simulink model "Main_SpeedOptimisedVersionTannenweg"  (R2024b)
settings: Solver=ode15s  StartTime=0.0  StopTime=3600*2  FixedStep=0.1  RelTol=0.001
model workspace (MAT data in the model file):
  Ti = 5
  fa = 0.00071
  fd = 0.03
  ips = 36
  ma = 0.0013
  md = 0.04
  roomarea1 = 20
  s = 15
libraries: fl_lib x1434, nesl_utility x105, SimscapeFluids_lib x35
(part 1 of 22)
settings Model: SimulationMode=accelerator  Creator=ferdi  LastModifiedBy=ferdi
settings SolverCC: MaxConsecutiveMinStep=5  ZeroCrossControl=EnableAll

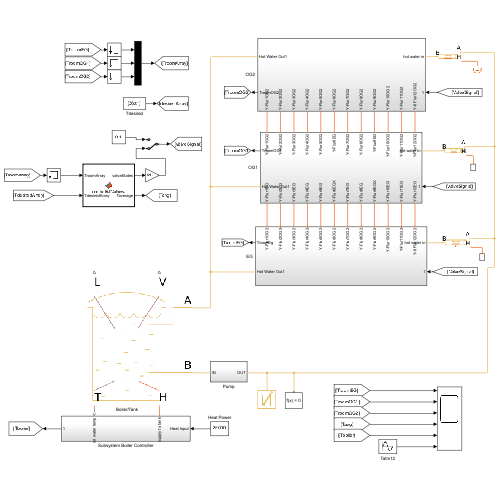
[thumbnail: Simulink's stored preview of the top-level diagram]
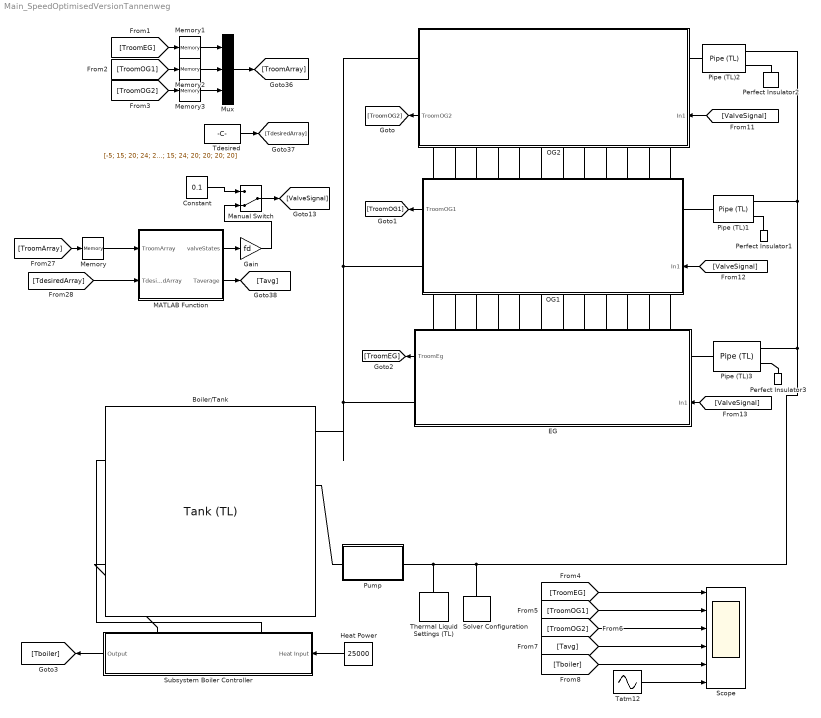
== system Main_SpeedOptimisedVersionTannenweg ==
  Boiler/Tank : SimscapeFluids_lib/Thermal Liquid/Tanks & Accumulators/Tank (TL)  num_inlet=fluids.thermal_liquid.tanks_accumulators.enum.NumInlet.Two  pressure_spec=fluids.thermal_liquid.tanks_accumulators.enum.TankPressureSpec.Atmospheric  tank_pressure=0.101325 MPa  volume_spec=fluids.thermal_liquid.tanks_accumulators.enum.TankVolumeSpec.Constant  tank_area=5 m^2  level_TLU=[0, 3, 5] m  volume_TLU=[0, 4, 6] m^3  inlet_height_A=0.1 m  inlet_area_A=0.01 m^2  inlet_heights_AB=[.1, .1] m  inlet_areas_AB=[ma, ma] m^2  inlet_heights_ABC=[.1, .1, .1] m  inlet_areas_ABC=[.01, .01, .01] m^2  inlet_heights_ABCD=0.1 * ones(1, 4) m  inlet_areas_ABCD=0.01 * ones(1, 4) m^2  inlet_heights_ABCDE=0.1 * ones(1, 5) m  inlet_areas_ABCDE=0.01 * ones(1, 5) m^2  inlet_heights_ABCDEF=0.1 * ones(1, 6) m  inlet_areas_ABCDEF=0.01 * ones(1, 6) m^2  level_check=simscape.enum.assert.action.error  capacity_check=simscape.enum.assert.action.none  max_capacity=10 m^3  g=9.81 m/s^2  level_specify=off  level_priority=High  level=5 m  level_nominal_specify=on  level_nominal_value=5  level_nominal_unit=m  volume_specify=on  volume_priority=None  volume=25 m^3  volume_nominal_specify=on  volume_nominal_value=27  volume_nominal_unit=m^3  mass_specify=on  mass_priority=None  mass=25000 kg  mass_nominal_specify=off  mass_nominal_value=1  mass_nominal_unit=kg  T_I_specify=on  T_I_priority=High  T_I=55 degC  T_I_nominal_specify=off  T_I_nominal_value=1  T_I_nominal_unit=K
      settings: InternalSimscapePortConfiguration="{\"Bottom\":[{\"id\":\"H\",\"label\":\"H\",\"type\":\"foundation.thermal.thermal\"},{\"id\":\"T_out\",\"label\":\"T\",\"type\":\"output\"}],\"Left\":[{\"id\":\"A\",\"label\":\"A\",\"type\":\"foundation.thermal_liquid.thermal_liquid\"},{\"id\":\"B\",\"label\":\"B\",\"type\":\"foundation.thermal_liquid.thermal_liquid\"}],\"Right\":[],\"Top\":[{\"id\":\"V_out\",\"label\":\"V\",\"type\":\"output\"},{\"id\":\"L_out\",\"label\":\"L\",\"type\":\"output\"}]}"
  Constant : Constant  Value=0.1
  EG : Subsystem
      settings: PortSchema="{\"entries\":[{\"content\":{\"sides\":[{\"content\":{\"connectorIds\":[\"In1\",\"LConn1\"]},\"type\":\"ConnectorPlacement.EquallySpacedRectSide\",\"uuid\":\"2656af94-fbaa-4cdb-8b28-cfd3398b16ef\"},{\"content\":{\"connectorIds\":[\"RConn1\",\"Out1\"],\"side\":\"RIGHT\"},\"type\":\"ConnectorPlacement.EquallySpacedRectSide\",\"uuid\":\"da923e50-de3a-407d-b440-bba41caa8d09\"},{\"content\":{\"side\":\"TOP\"},\"type\":\"ConnectorPlacement.EquallySpacedRectSide\",\"uuid\":\"d00b7d3b-fad0-43e7-8322-d8df48fa7e08\"},{\"content\":{\"connectorIds\":[\"RConn2\",\"RConn3\",\"RConn4\",\"RConn5\",\"RConn6\",\"RConn7\",\"RConn8\",\"RConn9\",\"RConn10\",\"RConn11\",\"RConn12\",\"RConn13\"],\"side\":\"BOTTOM\"},\"type\":\"ConnectorPlacement.EquallySpacedRectSide\",\"uuid\":\"2d6cf44f-790a-4efb-a1e3-b38be23d7dad\"}]},\"type\":\"ConnectorPlacement.EquallySpacedConnector\",\"uuid\":\"43b409cf-1277-4d86-ba4e-16516e35aeb3\"}],\"packageUris\":[\"http://schema.mathworks.com/mf0/Connector/R2020b\"],\"version\":\"1.0\"}"
  Gain : Gain  Gain=fd
  Heat Power : Constant  Value=25000
  MATLAB Function : MATLAB Function  TreatAsAtomicUnit=on
  Manual Switch : ManualSwitch  CurrentSetting=0
  Memory{,1..3} (4 alike) : Memory
  Mux : Mux  Inputs=3
  OG1 : Subsystem
      settings: PortSchema="{\"entries\":[{\"content\":{\"sides\":[{\"content\":{\"connectorIds\":[\"In1\",\"LConn1\"]},\"type\":\"ConnectorPlacement.EquallySpacedRectSide\",\"uuid\":\"2656af94-fbaa-4cdb-8b28-cfd3398b16ef\"},{\"content\":{\"connectorIds\":[\"RConn1\",\"Out1\"],\"side\":\"RIGHT\"},\"type\":\"ConnectorPlacement.EquallySpacedRectSide\",\"uuid\":\"da923e50-de3a-407d-b440-bba41caa8d09\"},{\"content\":{\"connectorIds\":[\"LConn2\",\"LConn3\",\"LConn4\",\"LConn5\",\"LConn6\",\"LConn7\",\"LConn8\",\"LConn9\",\"LConn10\",\"LConn11\",\"LConn12\",\"LConn13\"],\"side\":\"TOP\"},\"type\":\"ConnectorPlacement.EquallySpacedRectSide\",\"uuid\":\"d00b7d3b-fad0-43e7-8322-d8df48fa7e08\"},{\"content\":{\"connectorIds\":[\"RConn2\",\"RConn3\",\"RConn4\",\"RConn5\",\"RConn6\",\"RConn7\",\"RConn8\",\"RConn9\",\"RConn10\",\"RConn11\",\"RConn12\",\"RConn13\"],\"side\":\"BOTTOM\"},\"type\":\"ConnectorPlacement.EquallySpacedRectSide\",\"uuid\":\"2d6cf44f-790a-4efb-a1e3-b38be23d7dad\"}]},\"type\":\"ConnectorPlacement.EquallySpacedConnector\",\"uuid\":\"43b409cf-1277-4d86-ba4e-16516e35aeb3\"}],\"packageUris\":[\"http://schema.mathworks.com/mf0/Connector/R2020b\"],\"version\":\"1.0\"}"
  OG2 : Subsystem
      settings: PortSchema="{\"entries\":[{\"content\":{\"sides\":[{\"content\":{\"connectorIds\":[\"LConn1\",\"In1\"]},\"type\":\"ConnectorPlacement.EquallySpacedRectSide\",\"uuid\":\"2656af94-fbaa-4cdb-8b28-cfd3398b16ef\"},{\"content\":{\"connectorIds\":[\"RConn1\",\"Out1\"],\"side\":\"RIGHT\"},\"type\":\"ConnectorPlacement.EquallySpacedRectSide\",\"uuid\":\"da923e50-de3a-407d-b440-bba41caa8d09\"},{\"content\":{\"side\":\"TOP\"},\"type\":\"ConnectorPlacement.EquallySpacedRectSide\",\"uuid\":\"d00b7d3b-fad0-43e7-8322-d8df48fa7e08\"},{\"content\":{\"connectorIds\":[\"RConn2\",\"RConn3\",\"RConn4\",\"RConn5\",\"RConn6\",\"RConn7\",\"RConn8\",\"RConn9\",\"RConn10\",\"RConn11\",\"RConn12\",\"RConn13\"],\"side\":\"BOTTOM\"},\"type\":\"ConnectorPlacement.EquallySpacedRectSide\",\"uuid\":\"2d6cf44f-790a-4efb-a1e3-b38be23d7dad\"}]},\"type\":\"ConnectorPlacement.EquallySpacedConnector\",\"uuid\":\"43b409cf-1277-4d86-ba4e-16516e35aeb3\"}],\"packageUris\":[\"http://schema.mathworks.com/mf0/Connector/R2020b\"],\"version\":\"1.0\"}"
  Perfect Insulator1 : fl_lib/Thermal/Thermal Elements/Perfect Insulator  T_specify=off  T_priority=None  T=293.15 K  T_nominal_specify=off  T_nominal_value=1  T_nominal_unit=K
  Perfect Insulator2 : fl_lib/Thermal/Thermal Elements/Perfect Insulator  T_specify=off  T_priority=None  T=293.15 K  T_nominal_specify=off  T_nominal_value=1  T_nominal_unit=K
  Perfect Insulator3 : fl_lib/Thermal/Thermal Elements/Perfect Insulator  T_specify=off  T_priority=None  T=293.15 K  T_nominal_specify=off  T_nominal_value=1  T_nominal_unit=K
  Pipe (TL)1 : fl_lib/Thermal Liquid/Elements/Pipe (TL)  length=4.8 m  area=ma m^2  Dh=md m  length_add=1 m  roughness=15e-6 m  Re_lam=2000  Re_tur=4000  shape_factor=64  Nu_lam=3.66  dynamic_compressibility=true  inertia=false  p0=0.101325 MPa  T0=293.15 K  mdot0=0 kg/s
  Pipe (TL)2 : fl_lib/Thermal Liquid/Elements/Pipe (TL)  length=7.6 m  area=ma m^2  Dh=md m  length_add=1 m  roughness=15e-6 m  Re_lam=2000  Re_tur=4000  shape_factor=64  Nu_lam=3.66  dynamic_compressibility=true  inertia=false  p0=0.101325 MPa  T0=293.15 K  mdot0=0 kg/s
  Pipe (TL)3 : fl_lib/Thermal Liquid/Elements/Pipe (TL)  length=2 m  area=ma m^2  Dh=md m  length_add=1 m  roughness=15e-6 m  Re_lam=2000  Re_tur=4000  shape_factor=64  Nu_lam=3.66  dynamic_compressibility=true  inertia=false  p0=0.101325 MPa  T0=293.15 K  mdot0=0 kg/s
  Pump : Subsystem
      settings: PortSchema="{\"entries\":[{\"content\":{\"sides\":[{\"content\":{},\"type\":\"ConnectorPlacement.EquallySpacedRectSide\",\"uuid\":\"6c4af18d-f8fe-44c2-baba-c678dedb7514\"},{\"content\":{\"side\":\"RIGHT\"},\"type\":\"ConnectorPlacement.EquallySpacedRectSide\",\"uuid\":\"e67d3007-1da7-46b5-b3e8-302f65e107ea\"},{\"content\":{\"connectorIds\":[\"LConn1\"],\"side\":\"TOP\"},\"type\":\"ConnectorPlacement.EquallySpacedRectSide\",\"uuid\":\"e390c6ba-3993-4bdd-a4fa-a3ffec9d74f1\"},{\"content\":{\"connectorIds\":[\"RConn1\"],\"side\":\"BOTTOM\"},\"type\":\"ConnectorPlacement.EquallySpacedRectSide\",\"uuid\":\"a62ac90e-623e-483b-9a51-1fd62e714745\"}]},\"type\":\"ConnectorPlacement.EquallySpacedConnector\",\"uuid\":\"b6a4287e-aed5-4256-ab6a-ea8ae0115076\"}],\"packageUris\":[\"http://schema.mathworks.com/mf0/Connector/R2020b\"],\"version\":\"1.0\"}"
  Scope : Scope  NumInputPorts=6
  Solver Configuration : nesl_utility/Solver Configuration  PhysicalDomain=network_engine_domain  SubClassName=solver  LeftPortType=input  RightPortType=generic  Tones=[]  Harmonics=[]  SimulateNoise=off  Profile=off  UseLocalSampling=off  EnableSwitchedLinearOptims=on  FrequencyDomain=off  UseCCode=off  RelTol=0.001  AbsTol=0.001  MinStep=1e-09  ToWorkspace=off  RevertToSquareIcSolve=off  NumHomotopyIterations=100  PhasorMode=off  PhasorModeNumHarmonics=1  ConsistencySolver=NEWTON_XTOL_AFTER_FTOL  IndexReductionMethod=DerivativeReplacement  DoDC=off  ResidualTolerance=1e-09  ConsistencyTolSource=GLOBAL  ConsistencyAbsTol=0.001  ConsistencyRelTol=0.001  ConsistencyTolFactor=0.001  UseLocalSolver=off  LocalSolverChoice=NE_BACKWARD_EULER_ADVANCER  ResolveIndetEquations=on  FunctionEvalNumThread=1  LocalSolverSampleTime=0.001  DoFixedCost=off  MaxNonlinIter=3  MaxModeIter=2  ComputeImpulses=off  ImpulseIterations=2  LinearAlgebra=auto  LinearAlgebraNumThread=0  EquationFormulation=NE_TIME_EF  DelaysMemoryBudget=1024  AutomaticFiltering=on  FilteringTimeConstant=0.001  PartitionStorageMethod=AS_NEEDED  PartitionMemoryBudget=1024  PartitionMethod=ROBUST  MultibodyUseLocalSolver=off  MultibodyLocalSolverChoice=ODE1  MultibodyLocalSolverSampleTime=0.001
  Subsystem Boiler Controller : Subsystem
      settings: PortSchema="{\"entries\":[{\"content\":{\"sides\":[{\"content\":{\"connectorIds\":[\"In1\"]},\"type\":\"ConnectorPlacement.EquallySpacedRectSide\",\"uuid\":\"e7750da8-9cb3-4133-899c-c72a77ff6dd9\"},{\"content\":{\"connectorIds\":[\"Out1\"],\"side\":\"RIGHT\"},\"type\":\"ConnectorPlacement.EquallySpacedRectSide\",\"uuid\":\"07247844-436f-42d1-bf44-41b0acb7a571\"},{\"content\":{\"connectorIds\":[\"LConn1\",\"LConn2\"],\"side\":\"TOP\"},\"type\":\"ConnectorPlacement.EquallySpacedRectSide\",\"uuid\":\"d71ce214-d117-4844-8b18-b77bcc45f26b\"},{\"content\":{\"side\":\"BOTTOM\"},\"type\":\"ConnectorPlacement.EquallySpacedRectSide\",\"uuid\":\"a67a4664-f3b4-445e-bf57-56add1a19a7b\"}]},\"type\":\"ConnectorPlacement.EquallySpacedConnector\",\"uuid\":\"1154f811-4e57-4459-9411-93f66fb1d81b\"}],\"packageUris\":[\"http://schema.mathworks.com/mf0/Connector/R2020b\"],\"version\":\"1.0\"}"
  Tatm12 : Sin  Amplitude=7  Frequency=2*pi/(24*3600)  Phase=pi  SampleTime=0
  Tdesired : Constant  Value=[-5; 15; 20; 24; 20; 20; 15; 24; 20; 20; 20; 20; -5; 15; 20; 24; 20; 20; 15; 24; 20; 20; 20; 20; -5; 15; 20; 24; 20; 20; 15; 24; 20; 20; 20; 20]  VectorParams1D=off  LockScale=on
  Thermal Liquid Settings (TL) : fl_lib/Thermal Liquid/Utilities/Thermal Liquid Settings (TL)  table_dimensions=foundation.enum.table_dimensions_TL.two_dimensional  T_TLU=[273.1600 : 10 : 373.16]' K  p_TLU=[0.01, 0.1, 5 : 5 : 50] MPa  p_atm=0.101325 MPa  pT_region_flag=foundation.enum.pT_region_TL.min_max  T_min=273.16 K  T_max=363.16 K  p_min=0.05 MPa  p_max=50 MPa  T_min_1D=273.16 K  T_max_1D=363.16 K  p_min_1D=0.05 MPa  p_max_1D=50 MPa  pT_validity_TLU=[1, 1, 1, 1, 1, 1, 1, 1, 1, 1, 1, 1; 1, 1, 1, 1, 1, 1, 1, 1, 1, 1, 1, 1; 1, 1, 1, 1, 1, 1, 1, 1, 1, 1, 1, 1; 1, 1, 1, 1, 1, 1, 1, 1, 1, 1, 1, 1; 1, 1, 1, 1, 1, 1, 1, 1, 1, 1, 1, 1; 0, 1, 1, 1, 1, 1, 1, 1, 1, 1, 1, 1; 0, 1, 1, 1, 1, 1, 1, 1, 1, 1, 1, 1; 0, 1, 1, 1, 1, 1, 1, 1, 1, 1, 1, 1; 0, 1, 1, 1, 1, 1, 1, 1, 1, 1, 1, 1; 0, 1, 1, 1, 1, 1, 1, 1, 1, 1, 1, 1; 0, 0, 1, 1, 1, 1, 1, 1, 1, 1, 1, 1]  properties_range_check=simscape.enum.assert.action.error  rho_parameterization_2D=foundation.enum.rho_parameterization_2D.rho_beta_alpha  rho_parameterization_1D=foundation.enum.rho_parameterization_1D.rho_vector  rho_TLU=[999.7973, 999.8431, 1002.3216, 1004.8218, 1007.293, 1009.7358, 1012.1506, 1014.5379, 1016.8979, 1019.2311, 1021.538, 1023.8188; 999.6579, 999.7009, 1002.0303, 1004.382, 1006.7084, 1009.0101, 1011.2874, 1013.5407, 1015.7703, 1017.9766, 1020.1599, 1022.3206; 998.1632, 998.2045, 1000.4375, 1002.6924, 1004.9239, 1007.1324, 1009.3183, 1011.4819, 1013.6236, 1015.7438, 1017.8428, 1019.921; 995.6057, 995.6458, 997.8186, 1000.0128, 1002.1841, 1004.3332, 1006.4603, 1008.566, 1010.6505, 1012.7144, 1014.758, 1016.7815; 992.1724, 992.2119, 994.3513, 996.5113, 998.6484, 1000.7633, 1002.8563, 1004.928, 1006.9788, 1009.009, 1011.0192, 1013.0097; 988.02, 988.0299, 990.1568, 992.3035, 994.4268, 996.5273, 998.6056, 1000.6622, 1002.6976, 1004.7123, 1006.7067, 1008.6813; 983.18, 983.1901, 985.3217, 987.4721, 989.5983, 991.7008, 993.7803, 995.8374, 997.8726, 999.8864, 1001.8795, 1003.8522; 977.75, 977.7583, 979.9094, 982.0783, 984.2216, 986.34, 988.4343, 990.505, 992.5529, 994.5786, 996.5825, 998.5654; 971.77, 971.7836, 973.9673, 976.1678, 978.3409, 980.4876, 982.6087, 984.7049, 986.7768, 988.8254, 990.8511, 992.8545; 965.26, 965.3023, 967.5311, 969.7753, 971.9901, 974.1764, 976.3354, 978.4676, 980.5741, 982.6556, 984.7129, 986.7465; 958.62, 958.6315, 960.627, 962.9267, 965.1944, 967.4314, 969.6387, 971.8173, 973.9681, 976.0921, 978.19, 980.2628] kg/m^3  beta_TLU=[1.9649, 1.9654, 1.9929, 2.0213, 2.0499, 2.0787, 2.1078, 2.1372, 2.1668, 2.1966, 2.2268, 2.2572; 2.0913, 2.0918, 2.1191, 2.1471, 2.1752, 2.2036, 2.2322, 2.261, 2.2899, 2.3191, 2.3485, 2.3781; 2.1786, 2.1791, 2.2067, 2.235, 2.2634, 2.2919, 2.3206, 2.3494, 2.3784, 2.4075, 2.4367, 2.4661; 2.2332, 2.2337, 2.2619, 2.2908, 2.3197, 2.3487, 2.3778, 2.407, 2.4363, 2.4657, 2.4951, 2.5246; 2.26, 2.2605, 2.2895, 2.3191, 2.3487, 2.3784, 2.4081, 2.4378, 2.4675, 2.4973, 2.5272, 2.5571; 2.2638, 2.2638, 2.2936, 2.324, 2.3544, 2.3848, 2.4151, 2.4455, 2.4758, 2.5062, 2.5365, 2.5669; 2.2472, 2.2472, 2.2779, 2.3092, 2.3403, 2.3715, 2.4025, 2.4336, 2.4646, 2.4955, 2.5264, 2.5573; 2.214, 2.214, 2.2455, 2.2776, 2.3096, 2.3415, 2.3733, 2.405, 2.4367, 2.4683, 2.4998, 2.5313; 2.1668, 2.1668, 2.1992, 2.2321, 2.2649, 2.2976, 2.3301, 2.3626, 2.3949, 2.4272, 2.4593, 2.4914; 2.1081, 2.1081, 2.1413, 2.175, 2.2086, 2.2421, 2.2754, 2.3085, 2.3415, 2.3744, 2.4072, 2.4399; 2.0494, 2.0494, 2.0739, 2.1084, 2.1428, 2.177, 2.211, 2.2449, 2.2786, 2.3121, 2.3455, 2.3788] GPa  alpha_TLU=1e-4 * [-.679, -.676, -.49, -.307, -.13, .041, .206, .365, .519, .668, .811, .949; .878, .881, .998, 1.114, 1.227, 1.337, 1.445, 1.549, 1.651, 1.75, 1.846, 1.939; 2.068, 2.069, 2.141, 2.213, 2.283, 2.352, 2.42, 2.486, 2.551, 2.614, 2.676, 2.736; 3.034, 3.035, 3.074, 3.113, 3.152, 3.191, 3.229, 3.267, 3.305, 3.341, 3.377, 3.413; 3.855, 3.856, 3.87, 3.884, 3.899, 3.914, 3.93, 3.946, 3.961, 3.977, 3.993, 4.009; 4.578, 4.578, 4.572, 4.566, 4.562, 4.558, 4.555, 4.552, 4.55, 4.549, 4.548, 4.547; 5.233, 5.233, 5.209, 5.186, 5.165, 5.144, 5.125, 5.107, 5.09, 5.074, 5.059, 5.045; 5.84, 5.84, 5.801, 5.762, 5.725, 5.691, 5.657, 5.625, 5.595, 5.566, 5.538, 5.512; 6.414, 6.414, 6.36, 6.307, 6.256, 6.208, 6.161, 6.117, 6.074, 6.033, 5.994, 5.956; 6.967, 6.967, 6.898, 6.831, 6.766, 6.705, 6.646, 6.589, 6.535, 6.482, 6.432, 6.384; 7.519, 7.519, 7.423, 7.342, 7.264, 7.189, 7.118, 7.049, 6.983, 6.92, 6.859, 6.8] 1/K  rho_TLU_2=[999.7973, 999.8431, 1002.3216, 1004.8218, 1007.293, 1009.7358, 1012.1506, 1014.5379, 1016.8979, 1019.2311, 1021.538, 1023.8188; 999.6579, 999.7009, 1002.0303, 1004.382, 1006.7084, 1009.0101, 1011.2874, 1013.5407, 1015.7703, 1017.9766, 1020.1599, 1022.3206; 998.1632, 998.2045, 1000.4375, 1002.6924, 1004.9239, 1007.1324, 1009.3183, 1011.4819, 1013.6236, 1015.7438, 1017.8428, 1019.921; 995.6057, 995.6458, 997.81864, 1000.0128, 1002.1841, 1004.3332, 1006.4603, 1008.566, 1010.6505, 1012.7144, 1014.758, 1016.7815; 992.1724, 992.2119, 994.3513, 996.5113, 998.6484, 1000.7633, 1002.8563, 1004.928, 1006.9788, 1009.009, 1011.0192, 1013.0097; 988.02, 988.0299, 990.1568, 992.3035, 994.4268, 996.5273, 998.6056, 1000.6622, 1002.6976, 1004.7123, 1006.7067, 1008.6813; 983.18, 983.1901, 985.3217, 987.4721, 989.5983, 991.7008, 993.7803, 995.8374, 997.8726, 999.8864, 1001.8795, 1003.8522; 977.75, 977.7583, 979.9094, 982.0783, 984.2216, 986.34, 988.4343, 990.505, 992.5529, 994.5786, 996.5825, 998.5654; 971.77, 971.7836, 973.9673, 976.1678, 978.3409, 980.4876, 982.6087, 984.7049, 986.7768, 988.8254, 990.8511, 992.8545; 965.26, 965.3023, 967.5311, 969.7753, 971.9901, 974.1764, 976.3354, 978.4676, 980.5741, 982.6556, 984.7129, 986.7465; 958.62, 958.6315, 960.627, 962.9267, 965.1944, 967.4314, 969.6387, 971.8173, 973.9681, 976.0921, 978.19, 980.2628] kg/m^3  rho_ref_3=998.21 kg/m^3  T_ref_3=293.16 K  p_ref_3=0.101325 MPa  beta_const_3=2.1791 GPa  alpha_const_3=2.0691e-4 1/K  rho_TLU_4=[999.84; 999.7; 998.2; 995.65; 992.21; 988.03; 983.19; 977.76; 971.78; 965.3; 958.8] kg/m^3  beta_const_4=2.1791 GPa  p_ref_4=0.101325 MPa  rho_ref_5=998.21 kg/m^3  T_ref_5=293.16 K  p_ref_5=0.101325 MPa  beta_const_5=2.1791 GPa  alpha_const_5=2.0691e-4 1/K  u_parameterization_2D=foundation.enum.u_parameterization_2D.u_cp  u_parameterization_1D=foundation.enum.u_parameterization_1D.u  u_TLU=[.0002, .0018, .086, .1588, .219, .267, .3034, .3288, .3436, .3483, .3435, .3294; 42.062, 42.06, 41.935, 41.804, 41.668, 41.527, 41.382, 41.233, 41.081, 40.924, 40.763, 40.599; 83.953, 83.948, 83.651, 83.349, 83.049, 82.749, 82.451, 82.153, 81.856, 81.56, 81.265, 80.971; 125.77, 125.76, 125.31, 124.86, 124.41, 123.97, 123.53, 123.1, 122.68, 122.25, 121.84, 121.42; 167.57, 167.56, 166.96, 166.37, 165.79, 165.21, 164.65, 164.09, 163.54, 163, 162.46, 161.94; 209.36, 209.36, 208.63, 207.9, 207.19, 206.48, 205.79, 205.11, 204.45, 203.79, 203.14, 202.5; 251.19, 251.19, 250.33, 249.47, 248.62, 247.79, 246.98, 246.18, 245.39, 244.62, 243.86, 243.12; 293.06, 293.06, 292.07, 291.07, 290.1, 289.14, 288.2, 287.28, 286.38, 285.49, 284.62, 283.77; 334.99, 334.99, 333.86, 332.73, 331.63, 330.54, 329.48, 328.44, 327.41, 326.41, 325.43, 324.46; 377, 377, 375.73, 374.46, 373.22, 372, 370.81, 369.64, 368.5, 367.38, 366.27, 365.19; 419.01, 419.01, 417.69, 416.27, 414.89, 413.54, 412.21, 410.91, 409.64, 408.4, 407.17, 405.98] kJ/kg  cp_TLU=[4.2199, 4.2194, 4.1957, 4.1726, 4.1508, 4.13, 4.1103, 4.0916, 4.0738, 4.0569, 4.0408, 4.0254; 4.1955, 4.1951, 4.1769, 4.1592, 4.1422, 4.1259, 4.1103, 4.0954, 4.0812, 4.0676, 4.0545, 4.0421; 4.1843, 4.184, 4.169, 4.1543, 4.1401, 4.1264, 4.1133, 4.1007, 4.0885, 4.0768, 4.0656, 4.0548; 4.1801, 4.1798, 4.1667, 4.1538, 4.1413, 4.1293, 4.1177, 4.1064, 4.0956, 4.0851, 4.075, 4.0653; 4.1796, 4.1794, 4.1675, 4.1558, 4.1444, 4.1334, 4.1227, 4.1123, 4.1023, 4.0926, 4.0832, 4.0741; 4.1813, 4.1813, 4.1702, 4.1592, 4.1484, 4.138, 4.1279, 4.1181, 4.1086, 4.0993, 4.0903, 4.0816; 4.185, 4.185, 4.1742, 4.1636, 4.1532, 4.1432, 4.1334, 4.1239, 4.1146, 4.1056, 4.0969, 4.0884; 4.1901, 4.1901, 4.1795, 4.169, 4.1588, 4.1489, 4.1393, 4.1299, 4.1207, 4.1118, 4.1032, 4.0947; 4.1968, 4.1968, 4.1862, 4.1757, 4.1655, 4.1555, 4.1458, 4.1364, 4.1273, 4.1183, 4.1096, 4.1012; 4.2052, 4.2052, 4.1944, 4.1837, 4.1733, 4.1632, 4.1534, 4.1438, 4.1345, 4.1255, 4.1166, 4.108; 4.2136, 4.2136, 4.2045, 4.1935, 4.1828, 4.1724, 4.1623, 4.1524, 4.1429, 4.1335, 4.1245, 4.1157] kJ/(K*kg)  u_TLU_2=[.0002, .0018, .086, .1588, .219, .267, .3034, .3288, .3436, .3483, .3435, .3294; 42.062, 42.06, 41.935, 41.804, 41.668, 41.527, 41.382, 41.233, 41.081, 40.924, 40.763, 40.599; 83.953, 83.948, 83.651, 83.349, 83.049, 82.749, 82.451, 82.153, 81.856, 81.56, 81.265, 80.971; 125.77, 125.76, 125.31, 124.86, 124.41, 123.97, 123.53, 123.1, 122.68, 122.25, 121.84, 121.42; 167.57, 167.56, 166.96, 166.37, 165.79, 165.21, 164.65, 164.09, 163.54, 163, 162.46, 161.94; 209.36, 209.36, 208.63, 207.9, 207.19, 206.48, 205.79, 205.11, 204.45, 203.79, 203.14, 202.5; 251.19, 251.19, 250.33, 249.47, 248.62, 247.79, 246.98, 246.18, 245.39, 244.62, 243.86, 243.12; 293.06, 293.06, 292.07, 291.07, 290.1, 289.14, 288.2, 287.28, 286.38, 285.49, 284.62, 283.77; 334.99, 334.99, 333.86, 332.73, 331.63, 330.54, 329.48, 328.44, 327.41, 326.41, 325.43, 324.46; 377, 377, 375.73, 374.46, 373.22, 372, 370.81, 369.64, 368.5, 367.38, 366.27, 365.19; 419.01, 419.01, 417.69, 416.27, 414.89, 413.54, 412.21, 410.91, 409.64, 408.4, 407.17, 405.98] kJ/kg  cp_TLU_3=[4.2199, 4.2194, 4.1957, 4.1726, 4.1508, 4.13, 4.1103, 4.0916, 4.0738, 4.0569, 4.0408, 4.0254; 4.1955, 4.1951, 4.1769, 4.1592, 4.1422, 4.1259, 4.1103, 4.0954, 4.0812, 4.0676, 4.0545, 4.0421; 4.1843, 4.184, 4.169, 4.1543, 4.1401, 4.1264, 4.1133, 4.1007, 4.0885, 4.0768, 4.0656, 4.0548; 4.1801, 4.1798, 4.1667, 4.1538, 4.1413, 4.1293, 4.1177, 4.1064, 4.0956, 4.0851, 4.075, 4.0653; 4.1796, 4.1794, 4.1675, 4.1558, 4.1444, 4.1334, 4.1227, 4.1123, 4.1023, 4.0926, 4.0832, 4.0741; 4.1813, 4.1813, 4.1702, 4.1592, 4.1484, 4.138, 4.1279, 4.1181, 4.1086, 4.0993, 4.0903, 4.0816; 4.185, 4.185, 4.1742, 4.1636, 4.1532, 4.1432, 4.1334, 4.1239, 4.1146, 4.1056, 4.0969, 4.0884; 4.1901, 4.1901, 4.1795, 4.169, 4.1588, 4.1489, 4.1393, 4.1299, 4.1207, 4.1118, 4.1032, 4.0947; 4.1968, 4.1968, 4.1862, 4.1757, 4.1655, 4.1555, 4.1458, 4.1364, 4.1273, 4.1183, 4.1096, 4.1012; 4.2052, 4.2052, 4.1944, 4.1837, 4.1733, 4.1632, 4.1534, 4.1438, 4.1345, 4.1255, 4.1166, 4.108; 4.2136, 4.2136, 4.2045, 4.1935, 4.1828, 4.1724, 4.1623, 4.1524, 4.1429, 4.1335, 4.1245, 4.1157] kJ/(K*kg)  u_TLU_4=[.0018; 42.06; 83.948; 125.76; 167.56; 209.36; 251.19; 293.06; 334.99; 377; 418.01] kJ/kg  cp_TLU_5=[4.2199; 4.1955; 4.1843; 4.1801; 4.1796; 4.1813; 4.185; 4.1901; 4.1968; 4.2052; 4.2136] kJ/(K*kg)  nu_TLU=[1.7917, 1.7914, 1.7763, 1.7615, 1.7473, 1.7338, 1.7208, 1.7085, 1.6967, 1.6854, 1.6747, 1.6645; 1.3061, 1.3059, 1.2986, 1.2914, 1.2845, 1.2779, 1.2716, 1.2656, 1.2598, 1.2543, 1.2491, 1.2441; 1.0032, 1.0032, .9995, .9959, .9924, .9891, .9859, .9829, .9801, .9774, .9748, .9724; .8006, .8005, .7987, .797, .7953, .7937, .7922, .7908, .7894, .7881, .787, .7859; .6577, .6577, .657, .6562, .6555, .6548, .6543, .6537, .6532, .6528, .6523, .652; .553, .553, .5529, .5527, .5526, .5525, .5524, .5524, .5524, .5524, .5524, .5525; .4739, .4739, .4741, .4743, .4745, .4747, .475, .4753, .4755, .4758, .4762, .4765; .4127, .4127, .4131, .4135, .4139, .4143, .4148, .4152, .4157, .4162, .4167, .4172; .3643, .3643, .3648, .3654, .3659, .3665, .367, .3676, .3682, .3688, .3694, .37; .3254, .3254, .3261, .3267, .3273, .328, .3286, .3293, .3299, .3306, .3312, .3319; .2866, .2866, .2945, .2952, .2959, .2965, .2972, .2979, .2986, .2993, .3, .3007] mm^2/s  nu_TLU_2=[1.7917; 1.3061; 1.0032; .8006; .6577; .553; .4739; .4127; .3643; .3254; .2866] mm^2/s  k_TLU=[561.04, 561.09, 563.8, 566.56, 569.32, 572.08, 574.82, 577.54, 580.24, 582.92, 585.57, 588.18; 580.02, 580.07, 582.45, 584.88, 587.32, 589.75, 592.18, 594.61, 597.02, 599.42, 601.8, 604.16; 598.44, 598.48, 600.73, 603.03, 605.33, 607.64, 609.94, 612.24, 614.54, 616.82, 619.1, 621.36; 615.48, 615.52, 617.73, 620, 622.26, 624.54, 626.81, 629.07, 631.34, 633.6, 635.85, 638.09; 630.6, 630.64, 632.87, 635.15, 637.44, 639.72, 642.01, 644.29, 646.57, 648.84, 651.11, 653.36; 643.61, 643.61, 645.88, 648.21, 650.53, 652.86, 655.18, 657.51, 659.82, 662.14, 664.44, 666.74; 654.39, 654.39, 656.73, 659.12, 661.5, 663.89, 666.27, 668.65, 671.02, 673.38, 675.74, 678.09; 663.13, 663.13, 665.54, 668, 670.46, 672.91, 675.36, 677.8, 680.24, 682.67, 685.09, 687.5; 670.02, 670.02, 672.51, 675.05, 677.59, 680.12, 682.64, 685.16, 687.67, 690.17, 692.66, 695.14; 675.27, 675.27, 677.85, 680.48, 683.11, 685.73, 688.34, 690.94, 693.53, 696.11, 698.68, 701.24; 680.52, 680.52, 681.77, 684.5, 687.22, 689.94, 692.64, 695.34, 698.02, 700.69, 703.35, 706] mW/(K*m)  k_TLU_2=[561.04; 580.02; 598.44; 615.48; 630.6; 643.61; 654.39; 663.13; 670.02; 675.27; 680.52] mW/(K*m)
  wires:
  Heat Power/1 -> Subsystem Boiler Controller/1(Heat Input)
  [ValveSignal] -> EG/1(In1)
  [ValveSignal] -> OG1/1(In1)
  [ValveSignal] -> OG2/1(In1)
  [TroomArray] -> Memory/1
  [TdesiredArray] -> MATLAB Function/2(TdesiredArray)
  MATLAB Function/2(Taverage) -> [Tavg]
  Tdesired/1 -> [TdesiredArray]
  MATLAB Function/1(valveStates) -> Gain/1
  Mux/1 -> [TroomArray]
  OG2/1(TroomOG2) -> [TroomOG2]
  OG1/1(TroomOG1) -> [TroomOG1]
  EG/1(TroomEg) -> [TroomEG]
  [TroomOG2] -> Scope/3
  [TroomOG1] -> Scope/2
  [TroomEG] -> Scope/1
  [Tavg] -> Scope/4
  Subsystem Boiler Controller/1(Output) -> [Tboiler]
  [Tboiler] -> Scope/5
  Tatm12/1 -> Scope/6
  [TroomEG] -> Memory1/1
  [TroomOG1] -> Memory2/1
  [TroomOG2] -> Memory3/1
  Memory/1 -> MATLAB Function/1(TroomArray)
  Memory1/1 -> Mux/1
  Gain/1 -> Manual Switch/2
  Memory2/1 -> Mux/2
  Memory3/1 -> Mux/3
  Constant/1 -> Manual Switch/1
  Manual Switch/1 -> [ValveSignal]
  connections:
  Subsystem Boiler Controller/LConn1 -- Boiler/Tank/RConn1
  Boiler/Tank/RConn2 -- Subsystem Boiler Controller/LConn2
  Pump/RConn1 -- Boiler/Tank/LConn2
  OG2/RConn1 -- EG/RConn1 -- Boiler/Tank/LConn1 -- OG1/RConn1
  EG/RConn2 -- OG1/LConn2
  EG/RConn3 -- OG1/LConn3
  EG/RConn4 -- OG1/LConn4
  EG/RConn5 -- OG1/LConn5
  EG/RConn6 -- OG1/LConn6
  EG/RConn7 -- OG1/LConn7
  EG/RConn8 -- OG1/LConn8
  EG/RConn9 -- OG1/LConn9
  EG/RConn10 -- OG1/LConn10
  EG/RConn11 -- OG1/LConn11
  EG/RConn12 -- OG1/LConn12
  EG/RConn13 -- OG1/LConn13
  OG1/RConn2 -- OG2/RConn2
  OG1/RConn3 -- OG2/RConn3
  OG1/RConn4 -- OG2/RConn4
  OG1/RConn5 -- OG2/RConn5
  OG1/RConn6 -- OG2/RConn6
  OG1/RConn7 -- OG2/RConn7
  OG1/RConn8 -- OG2/RConn8
  OG1/RConn9 -- OG2/RConn9
  OG1/RConn10 -- OG2/RConn10
  OG1/RConn11 -- OG2/RConn11
  OG1/RConn12 -- OG2/RConn12
  OG1/RConn13 -- OG2/RConn13
  Pipe (TL)2/LConn2 -- Perfect Insulator2/LConn1
  Solver Configuration/RConn1 -- Pipe (TL)2/LConn1 -- Pipe (TL)1/LConn1 -- Pipe (TL)3/LConn1 -- Thermal Liquid Settings (TL)/RConn1 -- Pump/LConn1
  Pipe (TL)3/LConn2 -- Perfect Insulator3/LConn1
  Pipe (TL)3/RConn1 -- EG/LConn1
  Pipe (TL)1/LConn2 -- Perfect Insulator1/LConn1
  Pipe (TL)1/RConn1 -- OG1/LConn1
  Pipe (TL)2/RConn1 -- OG2/LConn1

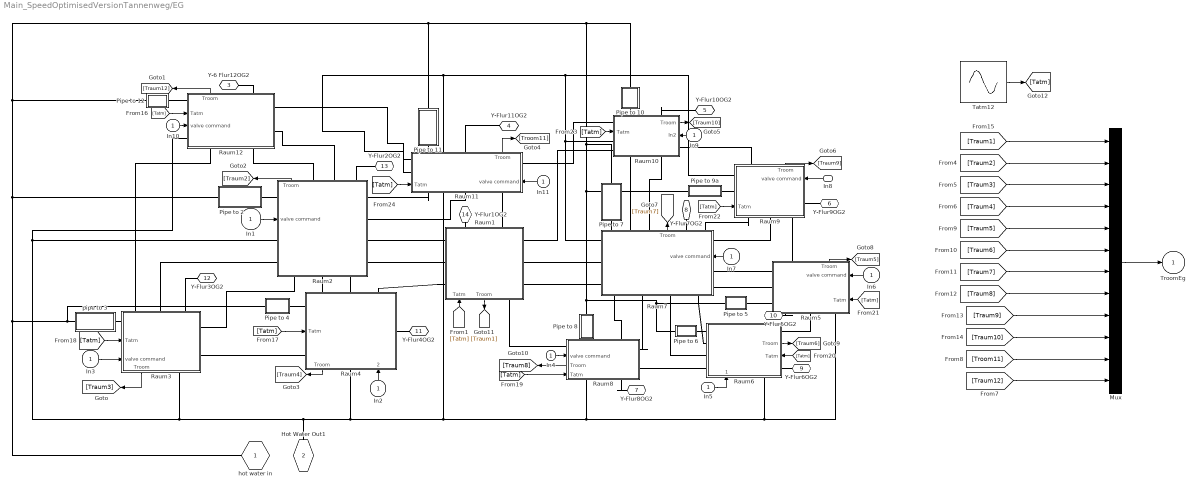
== system Main_SpeedOptimisedVersionTannenweg/EG ==
  In1 : Inport
  In{2..11} (10 alike) : InportShadow
  Mux : Mux  Inputs=12
  Pipe to 10 : Subsystem
  Pipe to 11 : Subsystem
  Pipe to 12 : Subsystem
  Pipe to 2 : Subsystem
  Pipe to 4 : Subsystem
  Pipe to 5 : Subsystem
  Pipe to 6 : Subsystem
  Pipe to 7 : Subsystem
  Pipe to 8 : Subsystem
  Pipe to 9a : Subsystem
  Raum1 : Subsystem
      settings: PortSchema="{\"entries\":[{\"content\":{\"sides\":[{\"content\":{\"connectorIds\":[\"LConn1\",\"LConn2\",\"LConn3\"]},\"type\":\"ConnectorPlacement.EquallySpacedRectSide\",\"uuid\":\"258852ae-79b4-4e90-ae22-4154c858ab0a\"},{\"content\":{\"connectorIds\":[\"RConn1\",\"RConn2\",\"RConn3\"],\"side\":\"RIGHT\"},\"type\":\"ConnectorPlacement.EquallySpacedRectSide\",\"uuid\":\"36706832-f330-42ce-9a32-f145cdee4912\"},{\"content\":{\"connectorIds\":[\"LConn4\",\"LConn5\"],\"side\":\"TOP\"},\"type\":\"ConnectorPlacement.EquallySpacedRectSide\",\"uuid\":\"5cf2347a-3520-447e-9561-2d1c8313f3cf\"},{\"content\":{\"connectorIds\":[\"RConn4\",\"Out1\",\"In1\"],\"side\":\"BOTTOM\"},\"type\":\"ConnectorPlacement.EquallySpacedRectSide\",\"uuid\":\"b1588268-8d41-4423-8f6e-2c28bf9b13dc\"}]},\"type\":\"ConnectorPlacement.EquallySpacedConnector\",\"uuid\":\"6bed35e7-1d7a-421b-a1f8-39267ed9017d\"}],\"packageUris\":[\"http://schema.mathworks.com/mf0/Connector/R2020b\"],\"version\":\"1.0\"}"
  Raum10 : Subsystem
      settings: PortSchema="{\"entries\":[{\"content\":{\"sides\":[{\"content\":{\"connectorIds\":[\"LConn1\",\"In1\",\"LConn2\",\"LConn3\"]},\"type\":\"ConnectorPlacement.EquallySpacedRectSide\",\"uuid\":\"258852ae-79b4-4e90-ae22-4154c858ab0a\"},{\"content\":{\"connectorIds\":[\"Out1\",\"In2\",\"RConn1\"],\"side\":\"RIGHT\"},\"type\":\"ConnectorPlacement.EquallySpacedRectSide\",\"uuid\":\"36706832-f330-42ce-9a32-f145cdee4912\"},{\"content\":{\"connectorIds\":[\"LConn4\",\"LConn5\"],\"side\":\"TOP\"},\"type\":\"ConnectorPlacement.EquallySpacedRectSide\",\"uuid\":\"5cf2347a-3520-447e-9561-2d1c8313f3cf\"},{\"content\":{\"connectorIds\":[\"RConn2\",\"RConn3\"],\"side\":\"BOTTOM\"},\"type\":\"ConnectorPlacement.EquallySpacedRectSide\",\"uuid\":\"b1588268-8d41-4423-8f6e-2c28bf9b13dc\"}]},\"type\":\"ConnectorPlacement.EquallySpacedConnector\",\"uuid\":\"6bed35e7-1d7a-421b-a1f8-39267ed9017d\"}],\"packageUris\":[\"http://schema.mathworks.com/mf0/Connector/R2020b\"],\"version\":\"1.0\"}"
  Raum11 : Subsystem
      settings: PortSchema="{\"entries\":[{\"content\":{\"sides\":[{\"content\":{\"connectorIds\":[\"LConn1\",\"LConn2\",\"In1\"]},\"type\":\"ConnectorPlacement.EquallySpacedRectSide\",\"uuid\":\"258852ae-79b4-4e90-ae22-4154c858ab0a\"},{\"content\":{\"connectorIds\":[\"RConn1\",\"In2\"],\"side\":\"RIGHT\"},\"type\":\"ConnectorPlacement.EquallySpacedRectSide\",\"uuid\":\"36706832-f330-42ce-9a32-f145cdee4912\"},{\"content\":{\"connectorIds\":[\"LConn3\",\"LConn4\",\"Out1\"],\"side\":\"TOP\"},\"type\":\"ConnectorPlacement.EquallySpacedRectSide\",\"uuid\":\"5cf2347a-3520-447e-9561-2d1c8313f3cf\"},{\"content\":{\"connectorIds\":[\"RConn2\",\"RConn3\",\"RConn4\"],\"side\":\"BOTTOM\"},\"type\":\"ConnectorPlacement.EquallySpacedRectSide\",\"uuid\":\"b1588268-8d41-4423-8f6e-2c28bf9b13dc\"}]},\"type\":\"ConnectorPlacement.EquallySpacedConnector\",\"uuid\":\"6bed35e7-1d7a-421b-a1f8-39267ed9017d\"}],\"packageUris\":[\"http://schema.mathworks.com/mf0/Connector/R2020b\"],\"version\":\"1.0\"}"
  Raum12 : Subsystem
      settings: PortSchema="{\"entries\":[{\"content\":{\"sides\":[{\"content\":{\"connectorIds\":[\"LConn1\",\"In1\",\"In2\",\"LConn2\"]},\"type\":\"ConnectorPlacement.EquallySpacedRectSide\",\"uuid\":\"258852ae-79b4-4e90-ae22-4154c858ab0a\"},{\"content\":{\"connectorIds\":[\"RConn1\",\"RConn2\"],\"side\":\"RIGHT\"},\"type\":\"ConnectorPlacement.EquallySpacedRectSide\",\"uuid\":\"36706832-f330-42ce-9a32-f145cdee4912\"},{\"content\":{\"connectorIds\":[\"Out1\",\"LConn3\"],\"side\":\"TOP\"},\"type\":\"ConnectorPlacement.EquallySpacedRectSide\",\"uuid\":\"5cf2347a-3520-447e-9561-2d1c8313f3cf\"},{\"content\":{\"connectorIds\":[\"RConn3\",\"RConn4\"],\"side\":\"BOTTOM\"},\"type\":\"ConnectorPlacement.EquallySpacedRectSide\",\"uuid\":\"b1588268-8d41-4423-8f6e-2c28bf9b13dc\"}]},\"type\":\"ConnectorPlacement.EquallySpacedConnector\",\"uuid\":\"6bed35e7-1d7a-421b-a1f8-39267ed9017d\"}],\"packageUris\":[\"http://schema.mathworks.com/mf0/Connector/R2020b\"],\"version\":\"1.0\"}"
  Raum2 : Subsystem
      settings: PortSchema="{\"entries\":[{\"content\":{\"sides\":[{\"content\":{\"connectorIds\":[\"LConn1\",\"In1\",\"LConn2\",\"LConn3\"]},\"type\":\"ConnectorPlacement.EquallySpacedRectSide\",\"uuid\":\"258852ae-79b4-4e90-ae22-4154c858ab0a\"},{\"content\":{\"connectorIds\":[\"RConn1\",\"RConn2\",\"RConn3\",\"RConn4\"],\"side\":\"RIGHT\"},\"type\":\"ConnectorPlacement.EquallySpacedRectSide\",\"uuid\":\"36706832-f330-42ce-9a32-f145cdee4912\"},{\"content\":{\"connectorIds\":[\"Out1\",\"LConn4\",\"LConn5\",\"LConn6\"],\"side\":\"TOP\"},\"type\":\"ConnectorPlacement.EquallySpacedRectSide\",\"uuid\":\"5cf2347a-3520-447e-9561-2d1c8313f3cf\"},{\"content\":{\"connectorIds\":[\"RConn5\",\"RConn6\",\"RConn7\"],\"side\":\"BOTTOM\"},\"type\":\"ConnectorPlacement.EquallySpacedRectSide\",\"uuid\":\"b1588268-8d41-4423-8f6e-2c28bf9b13dc\"}]},\"type\":\"ConnectorPlacement.EquallySpacedConnector\",\"uuid\":\"6bed35e7-1d7a-421b-a1f8-39267ed9017d\"}],\"packageUris\":[\"http://schema.mathworks.com/mf0/Connector/R2020b\"],\"version\":\"1.0\"}"
  Raum3 : Subsystem
      settings: PortSchema="{\"entries\":[{\"content\":{\"sides\":[{\"content\":{\"connectorIds\":[\"LConn1\",\"In1\",\"In2\"]},\"type\":\"ConnectorPlacement.EquallySpacedRectSide\",\"uuid\":\"258852ae-79b4-4e90-ae22-4154c858ab0a\"},{\"content\":{\"connectorIds\":[\"RConn1\",\"RConn2\"],\"side\":\"RIGHT\"},\"type\":\"ConnectorPlacement.EquallySpacedRectSide\",\"uuid\":\"36706832-f330-42ce-9a32-f145cdee4912\"},{\"content\":{\"connectorIds\":[\"LConn2\",\"LConn3\",\"LConn4\"],\"side\":\"TOP\"},\"type\":\"ConnectorPlacement.EquallySpacedRectSide\",\"uuid\":\"5cf2347a-3520-447e-9561-2d1c8313f3cf\"},{\"content\":{\"connectorIds\":[\"Out1\",\"RConn3\"],\"side\":\"BOTTOM\"},\"type\":\"ConnectorPlacement.EquallySpacedRectSide\",\"uuid\":\"b1588268-8d41-4423-8f6e-2c28bf9b13dc\"}]},\"type\":\"ConnectorPlacement.EquallySpacedConnector\",\"uuid\":\"6bed35e7-1d7a-421b-a1f8-39267ed9017d\"}],\"packageUris\":[\"http://schema.mathworks.com/mf0/Connector/R2020b\"],\"version\":\"1.0\"}"
  Raum4 : Subsystem
      settings: PortSchema="{\"entries\":[{\"content\":{\"sides\":[{\"content\":{\"connectorIds\":[\"LConn1\",\"In1\",\"LConn2\"]},\"type\":\"ConnectorPlacement.EquallySpacedRectSide\",\"uuid\":\"258852ae-79b4-4e90-ae22-4154c858ab0a\"},{\"content\":{\"connectorIds\":[\"RConn1\"],\"side\":\"RIGHT\"},\"type\":\"ConnectorPlacement.EquallySpacedRectSide\",\"uuid\":\"36706832-f330-42ce-9a32-f145cdee4912\"},{\"content\":{\"connectorIds\":[\"LConn3\",\"LConn4\",\"LConn5\"],\"side\":\"TOP\"},\"type\":\"ConnectorPlacement.EquallySpacedRectSide\",\"uuid\":\"5cf2347a-3520-447e-9561-2d1c8313f3cf\"},{\"content\":{\"connectorIds\":[\"Out1\",\"RConn2\",\"In2\"],\"side\":\"BOTTOM\"},\"type\":\"ConnectorPlacement.EquallySpacedRectSide\",\"uuid\":\"b1588268-8d41-4423-8f6e-2c28bf9b13dc\"}]},\"type\":\"ConnectorPlacement.EquallySpacedConnector\",\"uuid\":\"6bed35e7-1d7a-421b-a1f8-39267ed9017d\"}],\"packageUris\":[\"http://schema.mathworks.com/mf0/Connector/R2020b\"],\"version\":\"1.0\"}"
  Raum5 : Subsystem
      settings: PortSchema="{\"entries\":[{\"content\":{\"sides\":[{\"content\":{\"connectorIds\":[\"LConn1\",\"LConn2\",\"LConn3\"]},\"type\":\"ConnectorPlacement.EquallySpacedRectSide\",\"uuid\":\"258852ae-79b4-4e90-ae22-4154c858ab0a\"},{\"content\":{\"connectorIds\":[\"In1\",\"In2\"],\"side\":\"RIGHT\"},\"type\":\"ConnectorPlacement.EquallySpacedRectSide\",\"uuid\":\"36706832-f330-42ce-9a32-f145cdee4912\"},{\"content\":{\"connectorIds\":[\"LConn4\",\"Out1\"],\"side\":\"TOP\"},\"type\":\"ConnectorPlacement.EquallySpacedRectSide\",\"uuid\":\"5cf2347a-3520-447e-9561-2d1c8313f3cf\"},{\"content\":{\"connectorIds\":[\"RConn1\",\"RConn2\",\"RConn3\"],\"side\":\"BOTTOM\"},\"type\":\"ConnectorPlacement.EquallySpacedRectSide\",\"uuid\":\"b1588268-8d41-4423-8f6e-2c28bf9b13dc\"}]},\"type\":\"ConnectorPlacement.EquallySpacedConnector\",\"uuid\":\"6bed35e7-1d7a-421b-a1f8-39267ed9017d\"}],\"packageUris\":[\"http://schema.mathworks.com/mf0/Connector/R2020b\"],\"version\":\"1.0\"}"
  Raum6 : Subsystem
      settings: PortSchema="{\"entries\":[{\"content\":{\"sides\":[{\"content\":{\"connectorIds\":[\"LConn1\",\"LConn2\",\"LConn3\",\"LConn4\"]},\"type\":\"ConnectorPlacement.EquallySpacedRectSide\",\"uuid\":\"258852ae-79b4-4e90-ae22-4154c858ab0a\"},{\"content\":{\"connectorIds\":[\"RConn1\",\"Out1\",\"In2\",\"RConn2\"],\"side\":\"RIGHT\"},\"type\":\"ConnectorPlacement.EquallySpacedRectSide\",\"uuid\":\"36706832-f330-42ce-9a32-f145cdee4912\"},{\"content\":{\"side\":\"TOP\"},\"type\":\"ConnectorPlacement.EquallySpacedRectSide\",\"uuid\":\"5cf2347a-3520-447e-9561-2d1c8313f3cf\"},{\"content\":{\"connectorIds\":[\"In1\",\"RConn3\"],\"side\":\"BOTTOM\"},\"type\":\"ConnectorPlacement.EquallySpacedRectSide\",\"uuid\":\"b1588268-8d41-4423-8f6e-2c28bf9b13dc\"}]},\"type\":\"ConnectorPlacement.EquallySpacedConnector\",\"uuid\":\"6bed35e7-1d7a-421b-a1f8-39267ed9017d\"}],\"packageUris\":[\"http://schema.mathworks.com/mf0/Connector/R2020b\"],\"version\":\"1.0\"}"
  Raum7 : Subsystem
      settings: PortSchema="{\"entries\":[{\"content\":{\"sides\":[{\"content\":{\"connectorIds\":[\"LConn1\",\"LConn2\",\"LConn3\"]},\"type\":\"ConnectorPlacement.EquallySpacedRectSide\",\"uuid\":\"258852ae-79b4-4e90-ae22-4154c858ab0a\"},{\"content\":{\"connectorIds\":[\"RConn1\",\"In1\",\"RConn2\",\"RConn3\"],\"side\":\"RIGHT\"},\"type\":\"ConnectorPlacement.EquallySpacedRectSide\",\"uuid\":\"36706832-f330-42ce-9a32-f145cdee4912\"},{\"content\":{\"connectorIds\":[\"LConn4\",\"LConn5\",\"LConn6\",\"Out1\",\"LConn7\",\"LConn8\"],\"side\":\"TOP\"},\"type\":\"ConnectorPlacement.EquallySpacedRectSide\",\"uuid\":\"5cf2347a-3520-447e-9561-2d1c8313f3cf\"},{\"content\":{\"connectorIds\":[\"RConn4\",\"RConn5\",\"RConn6\",\"RConn7\"],\"side\":\"BOTTOM\"},\"type\":\"ConnectorPlacement.EquallySpacedRectSide\",\"uuid\":\"b1588268-8d41-4423-8f6e-2c28bf9b13dc\"}]},\"type\":\"ConnectorPlacement.EquallySpacedConnector\",\"uuid\":\"6bed35e7-1d7a-421b-a1f8-39267ed9017d\"}],\"packageUris\":[\"http://schema.mathworks.com/mf0/Connector/R2020b\"],\"version\":\"1.0\"}"
  Raum8 : Subsystem
      settings: PortSchema="{\"entries\":[{\"content\":{\"sides\":[{\"content\":{\"connectorIds\":[\"LConn1\",\"In1\",\"Out1\",\"In2\"]},\"type\":\"ConnectorPlacement.EquallySpacedRectSide\",\"uuid\":\"258852ae-79b4-4e90-ae22-4154c858ab0a\"},{\"content\":{\"connectorIds\":[\"RConn1\",\"RConn2\"],\"side\":\"RIGHT\"},\"type\":\"ConnectorPlacement.EquallySpacedRectSide\",\"uuid\":\"36706832-f330-42ce-9a32-f145cdee4912\"},{\"content\":{\"connectorIds\":[\"LConn2\",\"LConn3\"],\"side\":\"TOP\"},\"type\":\"ConnectorPlacement.EquallySpacedRectSide\",\"uuid\":\"5cf2347a-3520-447e-9561-2d1c8313f3cf\"},{\"content\":{\"connectorIds\":[\"RConn3\",\"RConn4\"],\"side\":\"BOTTOM\"},\"type\":\"ConnectorPlacement.EquallySpacedRectSide\",\"uuid\":\"b1588268-8d41-4423-8f6e-2c28bf9b13dc\"}]},\"type\":\"ConnectorPlacement.EquallySpacedConnector\",\"uuid\":\"6bed35e7-1d7a-421b-a1f8-39267ed9017d\"}],\"packageUris\":[\"http://schema.mathworks.com/mf0/Connector/R2020b\"],\"version\":\"1.0\"}"
  Raum9 : Subsystem
      settings: PortSchema="{\"entries\":[{\"content\":{\"sides\":[{\"content\":{\"connectorIds\":[\"LConn1\",\"LConn2\",\"In1\"]},\"type\":\"ConnectorPlacement.EquallySpacedRectSide\",\"uuid\":\"258852ae-79b4-4e90-ae22-4154c858ab0a\"},{\"content\":{\"connectorIds\":[\"In2\",\"RConn1\"],\"side\":\"RIGHT\"},\"type\":\"ConnectorPlacement.EquallySpacedRectSide\",\"uuid\":\"36706832-f330-42ce-9a32-f145cdee4912\"},{\"content\":{\"connectorIds\":[\"LConn3\",\"Out1\"],\"side\":\"TOP\"},\"type\":\"ConnectorPlacement.EquallySpacedRectSide\",\"uuid\":\"5cf2347a-3520-447e-9561-2d1c8313f3cf\"},{\"content\":{\"connectorIds\":[\"RConn2\",\"RConn3\",\"RConn4\"],\"side\":\"BOTTOM\"},\"type\":\"ConnectorPlacement.EquallySpacedRectSide\",\"uuid\":\"b1588268-8d41-4423-8f6e-2c28bf9b13dc\"}]},\"type\":\"ConnectorPlacement.EquallySpacedConnector\",\"uuid\":\"6bed35e7-1d7a-421b-a1f8-39267ed9017d\"}],\"packageUris\":[\"http://schema.mathworks.com/mf0/Connector/R2020b\"],\"version\":\"1.0\"}"
  Tatm12 : Sin  Amplitude=7  Frequency=2*pi/(24*3600)  Phase=pi  SampleTime=0
  pipe to 3 : Subsystem
  hot water in : PMIOPort  Side=Left
  Hot Water Out1 : PMIOPort  Port=2  Side=Right
  Y-6 Flur12OG2 : PMIOPort  Port=3  Side=Right
  Y-Flur11OG2 : PMIOPort  Port=4  Side=Right
  Y-Flur10OG2 : PMIOPort  Port=5  Side=Right
  Y-Flur9OG2 : PMIOPort  Port=6  Side=Right
  Y-Flur8OG2 : PMIOPort  Port=7  Side=Right
  Y-Flur7OG2 : PMIOPort  Port=8  Side=Right
  Y-Flur6OG2 : PMIOPort  Port=9  Side=Right
  Y-Flur5OG2 : PMIOPort  Port=10  Side=Right
  Y-Flur4OG2 : PMIOPort  Port=11  Side=Right
  Y-Flur3OG2 : PMIOPort  Port=12  Side=Right
  Y-Flur2OG2 : PMIOPort  Port=13  Side=Right
  Y-Flur1OG2 : PMIOPort  Port=14  Side=Right
  TroomEg : Outport
  wires:
  Raum9/1(Troom) -> [Traum9]
  [Tatm] -> Raum11/1(Tatm)
  Raum6/1(Troom) -> [Traum6]
  [Tatm] -> Raum9/1(Tatm)
  Raum7/1(Troom) -> [Traum7]
  Raum11/1(Troom) -> [Troom11]
  Raum2/1(Troom) -> [Traum2]
  [Tatm] -> Raum10/1(Tatm)
  [Tatm] -> Raum1/1(Tatm)
  [Tatm] -> Raum5/2(Tatm)
  [Tatm] -> Raum3/1(Tatm)
  [Tatm] -> Raum4/1(Tatm)
  Raum3/1(Troom) -> [Traum3]
  Raum10/1(Troom) -> [Traum10]
  Raum1/1(Troom) -> [Traum1]
  [Tatm] -> Raum6/2(Tatm)
  [Tatm] -> Raum8/2(Tatm)
  Raum4/1(Troom) -> [Traum4]
  Raum5/1(Troom) -> [Traum5]
  Raum8/1(Troom) -> [Traum8]
  Raum12/1(Troom) -> [Traum12]
  [Tatm] -> Raum12/1(Tatm)
  Tatm12/1 -> [Tatm]
  In10/1 -> Raum12/2(valve command)
  In1/1 -> Raum2/1(valve command)
  In3/1 -> Raum3/2(valve command)
  In2/1 -> Raum4/2(valve command)
  In4/1 -> Raum8/1(valve command)
  In5/1 -> Raum6/1(valve command)
  In6/1 -> Raum5/1(valve command)
  In7/1 -> Raum7/1(valve command)
  In8/1 -> Raum9/2(valve command)
  In9/1 -> Raum10/2(In2)
  In11/1 -> Raum11/2(valve command)
  [Traum9] -> Mux/9
  [Traum7] -> Mux/7
  [Traum8] -> Mux/8
  [Traum12] -> Mux/12
  [Traum5] -> Mux/5
  [Traum6] -> Mux/6
  [Traum3] -> Mux/3
  [Traum4] -> Mux/4
  Mux/1 -> TroomEg/1
  [Traum2] -> Mux/2
  [Traum1] -> Mux/1
  [Troom11] -> Mux/11
  [Traum10] -> Mux/10
  connections:
  Raum6/LConn4 -- Raum8/RConn2
  Raum3/RConn3 -- Raum2/LConn2 -- Raum12/LConn2 -- Raum4/RConn2 -- Raum11/LConn1 -- Raum7/LConn1 -- Raum10/LConn2 -- Raum9/LConn1 -- Raum5/RConn3 -- Raum6/RConn3 -- Raum8/RConn3 -- Hot Water Out1/RConn1
  Raum5/RConn2 -- Raum6/RConn1
  Raum7/RConn6 -- Raum6/LConn3
  Pipe to 6/RConn1 -- Raum6/LConn1
  Raum1/RConn2 -- Raum2/RConn4
  Pipe to 12/RConn1 -- Raum12/LConn1
  Pipe to 7/RConn1 -- Raum7/LConn4
  Raum11/LConn2 -- Raum12/RConn1
  Raum3/LConn3 -- Raum2/LConn3
  Raum4/LConn4 -- Raum2/RConn7
  Raum11/RConn4 -- Raum1/LConn4
  Raum9/LConn2 -- Pipe to 9a/RConn1
  Raum5/LConn4 -- Raum9/RConn4
  Pipe to 4/RConn1 -- Raum4/LConn1
  Raum7/RConn7 -- Raum6/LConn2
  Pipe to 8/RConn1 -- Raum8/LConn2
  Pipe to 11/RConn1 -- Raum11/LConn3
  Raum9/RConn3 -- Raum7/RConn1
  Raum10/LConn1 -- Raum11/RConn1
  Raum2/LConn5 -- Raum12/RConn2
  Raum7/LConn3 -- Raum1/LConn3
  Pipe to 10/RConn1 -- Raum10/LConn4
  pipe to 3/RConn1 -- Raum3/LConn1
  Raum1/RConn4 -- Raum8/LConn1
  Raum9/LConn3 -- Raum10/RConn1
  Raum5/LConn2 -- Raum7/RConn3
  Raum2/RConn6 -- Raum4/LConn3
  Raum7/RConn4 -- Raum8/LConn3
  Raum3/LConn2 -- Raum12/RConn3
  Raum10/LConn3 -- Raum1/LConn1
  Pipe to 2/RConn1 -- Raum2/LConn1
  Raum12/RConn4 -- Raum2/LConn4
  Raum10/RConn3 -- Raum7/LConn6
  Raum7/RConn2 -- Raum5/LConn1
  Raum11/RConn2 -- Raum2/RConn1
  Raum3/RConn1 -- Raum2/RConn5
  Raum9/RConn2 -- Raum7/LConn8
  Raum3/RConn2 -- Raum4/LConn2
  Pipe to 5/RConn1 -- Raum5/LConn3
  Raum1/RConn3 -- Raum4/LConn5
  Raum1/LConn2 -- Raum7/LConn2
  Raum11/RConn3 -- Raum2/RConn2
  Raum8/RConn1 -- Raum7/RConn5
  Raum7/LConn5 -- Raum10/RConn2
  Raum2/RConn3 -- Raum1/RConn1
  Raum12/LConn3 -- Y-6 Flur12OG2/RConn1
  Raum11/LConn4 -- Y-Flur11OG2/RConn1
  Raum10/LConn5 -- Y-Flur10OG2/RConn1
  Raum9/RConn1 -- Y-Flur9OG2/RConn1
  Y-Flur5OG2/RConn1 -- Raum5/RConn1
  Raum7/LConn7 -- Y-Flur7OG2/RConn1
  Y-Flur6OG2/RConn1 -- Raum6/RConn2
  Y-Flur8OG2/RConn1 -- Raum8/RConn4
  Raum1/LConn5 -- Y-Flur1OG2/RConn1
  Y-Flur4OG2/RConn1 -- Raum4/RConn1
  Raum3/LConn4 -- Y-Flur3OG2/RConn1
  Raum2/LConn6 -- Y-Flur2OG2/RConn1
  hot water in/RConn1 -- pipe to 3/LConn1 -- Pipe to 4/LConn1 -- Pipe to 9a/LConn1 -- Pipe to 8/LConn1 -- Pipe to 6/LConn1 -- Pipe to 5/LConn1 -- Pipe to 7/LConn1 -- Pipe to 10/LConn1 -- Pipe to 11/LConn1 -- Pipe to 12/LConn1 -- Pipe to 2/LConn1
